simulink model "rocket_rcs"  (R2024a)
settings: Solver=FixedStepAuto  StartTime=0.0001  StopTime=140  FixedStep=0.0001  RelTol=1e-3
undefined symbols (not defined in the file or in its folder): deg, Earth, rad, s, WGS84
libraries: aerolibconvert2 x26, matrix_library x5, eePwmGenerator x5, slpidlib x5, aerolibasang x2, simulink x2, sharedtransform x1, aerolibtransform2 x1, shared6dof x1
(part 1 of 2)
settings Model: NumberOfSteps=10  Creator=WuZP  LastModifiedBy=WuZP

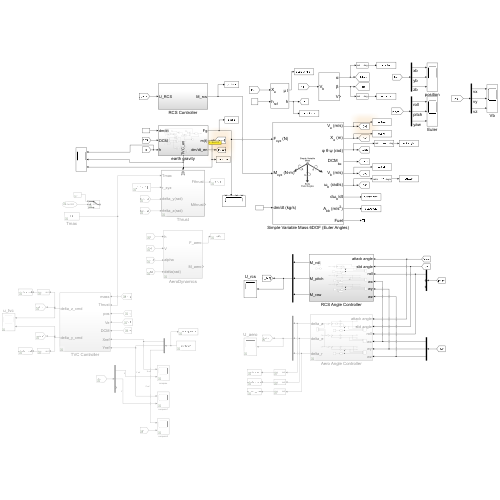
[thumbnail: Simulink's stored preview of the top-level diagram]
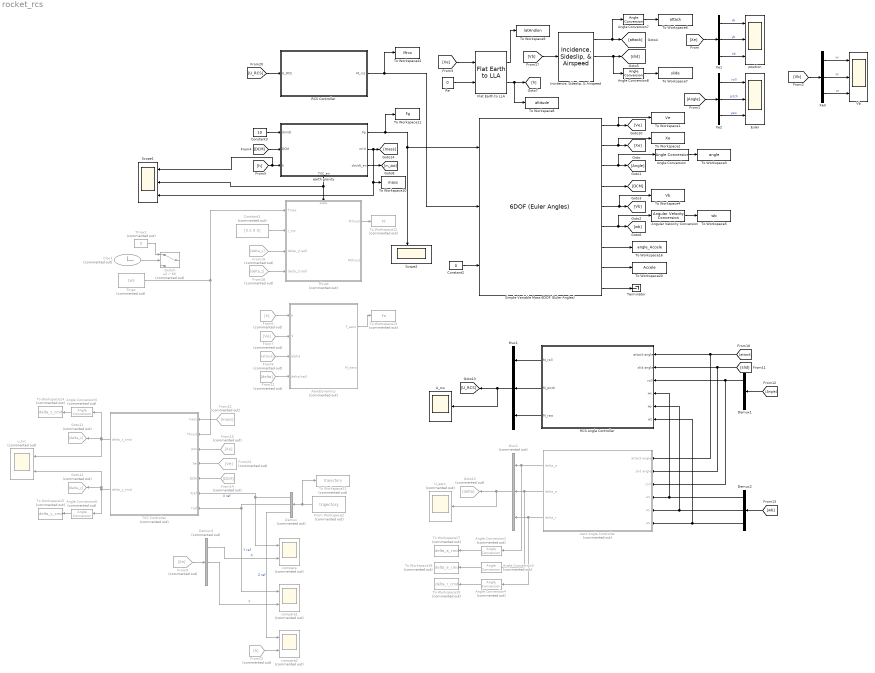
== system rocket_rcs ==
  Aero Angle Controller : Subsystem  Commented=on
  AeroDynamics : Subsystem  Commented=on
  Angle Conversion : aerolibconvert2/Angle Conversion  IU=rad  OU=deg
  Angle Conversion{2..6} (5 alike) : aerolibconvert2/Angle Conversion  Commented=on  IU=rad  OU=deg
  Angle Conversion7 : aerolibconvert2/Angle Conversion  IU=rad  OU=deg
  Angle Conversion8 : aerolibconvert2/Angle Conversion  IU=rad  OU=deg
  Angular Velocity Conversion : aerolibconvert2/Angular Velocity Conversion  IU=rad/s  OU=deg/s
  Clock : Clock  Commented=on
  Constant1 : Constant  Commented=on  Value=[3.5 0 0]
  Constant2 : Constant  Value=0
  Constant3 : Constant  Value=10
  Demux : Demux  Commented=on  Outputs=3
  Demux1 : Demux  Outputs=3
  Demux2 : Demux  Outputs=3
  Demux3 : Demux  Commented=on  Outputs=3
  Euler : Scope  NumInputPorts=3
  Flat Earth to LLA : aerolibtransform2/Flat Earth to LLA  units=Metric (MKS)  ptype=Earth (WGS84)  F=1/298.257223563  R=6378137  refPosPort=off  LL0=[39.73 98.49]  psi=0
  From Workspace2 : FromWorkspace  Commented=on  VariableName=trajectory
  From14 : From  Commented=on  GotoTag=DCM
  From15 : From  Commented=on  GotoTag=Xe
  From18 : From  Commented=on  GotoTag=delta_z
  From19 : From  Commented=on  GotoTag=delta_y
  From21 : From  Commented=on  GotoTag=mass
  From22 : From  Commented=on  GotoTag=delta
  From23 : From  Commented=on  GotoTag=h
  From24 : From  Commented=on  GotoTag=Ve
  From6 : From  Commented=on  GotoTag=h
  From7 : From  Commented=on  GotoTag=Ve
  From8 : From  Commented=on  GotoTag=attack
  From9 : From  Commented=on  GotoTag=Xe
  Goto11 : Goto  Commented=on  GotoTag=delta_z
  Goto12 : Goto  Commented=on  GotoTag=delta_y
  Goto15 : Goto  Commented=on  GotoTag=delta
  "Incidence, Sideslip, & Airspeed" : aerolibasang/Incidence, Sideslip, & Airspeed
  Mux1 : Mux  Inputs=3
  Mux2 : Mux  Commented=on  Inputs=3
  RCS Angle Controller : Subsystem
  RCS Controller : Subsystem
  Re : Constant  Value=0
  Scope1 : Scope  NumInputPorts=3
  Scope2 : Scope  NumInputPorts=4
  Simple Variable Mass 6DOF (Euler Angles) : shared6dof/6DOF (Euler Angles)  units=Metric (MKS)  mtype=Simple Variable  rep=Euler Angles  xme_0=[40719.4 121.1 -120000]  Vm_0=[7900 0 0]  eul_0=[0 0 0]  pm_0=[0 0 0]  mass_0=3600  mass_e=3600  mass_f=5000  inertia=eye(3)  inertia_e=eye(3)  inertia_f=2*eye(3)  k_quat=1.0  vre_flag=off  abi_flag=off  aMode=0  xme_statename=''  Vm_statename=''  eul_statename=''  quat_statename=''  pm_statename=''  mass_statename=''
      settings: LibrarySourceBlock=aerolib6dof2/Simple Variable Mass 6DOF (Euler Angles)
  Switch : Switch  Commented=on  Criteria=u2 > Threshold  Threshold=60  SaturateOnIntegerOverflow=off  InputSameDT=off
  TVC Controller : Subsystem  Commented=on
  Terminator : Terminator
  Thrust : Subsystem  Commented=on
  Tmax : Constant  Commented=on  Value=1e5
  Tmax1 : Constant  Commented=on  Value=0
  To Workspace1 : ToWorkspace  VariableName=Ve  SaveFormat=Timeseries  SampleTime=-1
  To Workspace10 : ToWorkspace  VariableName=mass  SaveFormat=Timeseries  SampleTime=-1
  To Workspace11 : ToWorkspace  VariableName=Fg  SaveFormat=Timeseries  SampleTime=-1
  To Workspace12 : ToWorkspace  Commented=on  VariableName=Ft  SaveFormat=Timeseries  SampleTime=-1
  To Workspace13 : ToWorkspace  Commented=on  VariableName=Fa  SaveFormat=Timeseries  SampleTime=-1
  To Workspace14 : ToWorkspace  Commented=on  VariableName=delta_z_cmd  SaveFormat=Timeseries  SampleTime=-1
  To Workspace15 : ToWorkspace  Commented=on  VariableName=delta_y_cmd  SaveFormat=Timeseries  SampleTime=-1
  To Workspace16 : ToWorkspace  VariableName=angle_Accele  SaveFormat=Timeseries  SampleTime=-1
  To Workspace17 : ToWorkspace  Commented=on  VariableName=delta_a_cmd  SaveFormat=Timeseries  SampleTime=-1
  To Workspace18 : ToWorkspace  Commented=on  VariableName=delta_e_cmd  SaveFormat=Timeseries  SampleTime=-1
  To Workspace19 : ToWorkspace  Commented=on  VariableName=delta_r_cmd  SaveFormat=Timeseries  SampleTime=-1
  To Workspace2 : ToWorkspace  VariableName=Xe  SaveFormat=Timeseries  SampleTime=-1
  To Workspace20 : ToWorkspace  VariableName=Accele  SaveFormat=Timeseries  SampleTime=-1
  To Workspace21 : ToWorkspace  Commented=on  VariableName=trajectory  SaveFormat=Timeseries  SampleTime=-1
  To Workspace22 : ToWorkspace  VariableName=Mrcs  SaveFormat=Timeseries  SampleTime=-1
  To Workspace3 : ToWorkspace  VariableName=angle  SaveFormat=Timeseries  SampleTime=-1
  To Workspace4 : ToWorkspace  VariableName=Vb  SaveFormat=Timeseries  SampleTime=-1
  To Workspace5 : ToWorkspace  VariableName=wb  SaveFormat=Timeseries  SampleTime=-1
  To Workspace6 : ToWorkspace  VariableName=attack  SaveFormat=Timeseries  SampleTime=-1
  To Workspace7 : ToWorkspace  VariableName=slide  SaveFormat=Timeseries  SampleTime=-1
  To Workspace8 : ToWorkspace  VariableName=altitude  SaveFormat=Timeseries  SampleTime=-1
  To Workspace9 : ToWorkspace  VariableName=latAndlon  SaveFormat=Timeseries  SampleTime=-1
  U_aero : Scope  Commented=on
  U_rcs : Scope
  Vb : Scope  NumInputPorts=3
  Xe1 : Demux  Outputs=3
  Xe2 : Demux  Outputs=3
  Xe3 : Demux  Outputs=3
  compare : Scope  Commented=on  NumInputPorts=2
  compare1 : Scope  Commented=on  NumInputPorts=2
  compare2 : Scope  Commented=on  NumInputPorts=2
  earth gravity : Subsystem
      settings: PortSchema="{\"entries\":[{\"content\":{\"sides\":[{\"content\":{\"connectorIds\":[\"In1\",\"In2\",\"In3\"]},\"type\":\"ConnectorPlacement.EquallySpacedRectSide\",\"uuid\":\"11dd11d9-77ad-45ee-ae63-619479f6c53b\"},{\"content\":{\"connectorIds\":[\"Out1\",\"Out2\",\"Out3\"],\"side\":\"RIGHT\"},\"type\":\"ConnectorPlacement.EquallySpacedRectSide\",\"uuid\":\"b6f331d1-51e3-4d01-85e1-3b5c4bfb552a\"},{\"content\":{\"side\":\"TOP\"},\"type\":\"ConnectorPlacement.EquallySpacedRectSide\",\"uuid\":\"4dab32ce-cfd7-4c7f-b135-3e557b532ba2\"},{\"content\":{\"connectorIds\":[\"Out4\"],\"side\":\"BOTTOM\"},\"type\":\"ConnectorPlacement.EquallySpacedRectSide\",\"uuid\":\"e34d9b96-68fb-4d6e-a900-086bc6e7115e\"}]},\"type\":\"ConnectorPlacement.EquallySpacedConnector\",\"uuid\":\"c83bfd2c-4554-412a-969b-4a26b6e2370b\"}],\"packageUris\":[\"http://schema.mathworks.com/mf0/Connector/R2020b\"],\"version\":\"1.0\"}"
  position : Scope  NumInputPorts=3
  u_tvc : Scope  Commented=on  NumInputPorts=2
  wires:
  Re/1 -> Flat Earth to LLA/2
  Tmax/1 -> Thrust/1(Tmax), TVC Controller/2(Thrust)
  Simple Variable Mass 6DOF (Euler Angles)/2 -> To Workspace2/1, [Xe]
  TVC Controller/1(delta_z_cmd) -> Angle Conversion5/1, Goto11/1, u_tvc/1
  Xe1/1 -> position/1  "xb"
  Xe1/2 -> position/2  "yb"
  Xe1/3 -> position/3  "zb"
  Simple Variable Mass 6DOF (Euler Angles)/3 -> Angle Conversion/1, [Angle]
  TVC Controller/2(delta_y_cmd) -> Goto12/1, u_tvc/2, Angle Conversion6/1
  From Workspace2/1 -> To Workspace21/1, Demux/1
  Demux/1 -> compare/1, TVC Controller/6(Xref)  "X ref"
  Demux/2 -> compare1/1, TVC Controller/7(Yref)  "Y ref"
  Constant3/1 -> earth gravity/1(dm/dt)
  Constant2/1 -> Simple Variable Mass 6DOF (Euler Angles)/3
  Simple Variable Mass 6DOF (Euler Angles)/5 -> To Workspace4/1, [Vb]
  "Incidence, Sideslip, & Airspeed"/1 -> Angle Conversion7/1, [attack]
  Xe3/3 -> Vb/3  "vz"
  Xe3/2 -> Vb/2  "vy"
  Xe3/1 -> Vb/1  "vx"
  "Incidence, Sideslip, & Airspeed"/2 -> Angle Conversion8/1, [slid]
  RCS Angle Controller/1(M_roll) -> Mux1/1
  RCS Angle Controller/2(M_pitch) -> Mux1/2
  RCS Angle Controller/3(M_raw) -> Mux1/3
  Aero Angle Controller/2(delta_e) -> Angle Conversion3/1, Mux2/2
  Aero Angle Controller/3(delta_r) -> Angle Conversion4/1, Mux2/3
  Aero Angle Controller/1(delta_a) -> Angle Conversion2/1, Mux2/1
  Mux2/1 -> Goto15/1, U_aero/1
  [Xe] -> Xe1/1
  [Vb] -> Xe3/1
  [Angle] -> Xe2/1
  Xe2/1 -> Euler/1  "roll"
  Xe2/2 -> Euler/2  "pitch"
  Xe2/3 -> Euler/3  "yaw"
  Simple Variable Mass 6DOF (Euler Angles)/4 -> [DCM]
  [Xe] -> Flat Earth to LLA/1
  Flat Earth to LLA/2 -> To Workspace8/1, [h]
  [DCM] -> earth gravity/2(DCM)
  [h] -> Scope1/1, earth gravity/3(h)
  From6/1 -> AeroDynamics/1(h)
  From7/1 -> AeroDynamics/2(V)
  From8/1 -> AeroDynamics/3(alpha)
  [attack] -> Aero Angle Controller/1(attack angle), RCS Angle Controller/1(attack angle)
  [slid] -> RCS Angle Controller/2(slid angle), Aero Angle Controller/2(slid angle)
  [Angle] -> Demux1/1
  Demux1/1 -> RCS Angle Controller/3(roll), Aero Angle Controller/3(roll)
  [wb] -> Demux2/1
  From14/1 -> TVC Controller/5(DCM)
  From15/1 -> TVC Controller/3(pos)
  Simple Variable Mass 6DOF (Euler Angles)/1 -> To Workspace1/1, [Ve]
  Constant1/1 -> Thrust/2(r_xyz)
  Simple Variable Mass 6DOF (Euler Angles)/9 -> Terminator/1
  Simple Variable Mass 6DOF (Euler Angles)/8 -> To Workspace20/1
  Simple Variable Mass 6DOF (Euler Angles)/7 -> To Workspace16/1
  [Vb] -> "Incidence, Sideslip, & Airspeed"/1
  earth gravity/4(TVC_en) -> Scope1/2, Thrust/Enable
  Mux1/1 -> [U_RCS], U_rcs/1
  [U_RCS] -> RCS Controller/1(U_RCS)
  earth gravity/2(m(t)) -> To Workspace10/1, Scope1/3, [mass]
  From21/1 -> TVC Controller/1(mass)
  From22/1 -> AeroDynamics/4(delta(rad))
  Demux2/1 -> RCS Angle Controller/4(wx), Aero Angle Controller/4(wx)
  Demux2/2 -> RCS Angle Controller/5(wy), Aero Angle Controller/5(wy)
  Demux2/3 -> RCS Angle Controller/6(wz), Aero Angle Controller/6(wz)
  Thrust/1(Fthrust) -> To Workspace12/1
  earth gravity/1(Fg) -> To Workspace11/1, Simple Variable Mass 6DOF (Euler Angles)/1, Scope2/2
  From19/1 -> Thrust/3(delta_y(rad))
  From18/1 -> Thrust/4(delta_z(rad))
  AeroDynamics/1(F_aero) -> To Workspace13/1
  From9/1 -> Demux3/1
  Demux3/1 -> compare/2  "X"
  Demux3/2 -> compare1/2  "Y"
  earth gravity/3(dm/dt_en) -> [m_dot]
  Demux/3 -> compare2/1  "Z ref"
  From23/1 -> compare2/2
  Flat Earth to LLA/1 -> To Workspace9/1
  Angle Conversion/1 -> To Workspace3/1
  Simple Variable Mass 6DOF (Euler Angles)/6 -> Angular Velocity Conversion/1, [wb]
  Angle Conversion2/1 -> To Workspace17/1
  Angle Conversion4/1 -> To Workspace19/1
  Angle Conversion3/1 -> To Workspace18/1
  Angle Conversion5/1 -> To Workspace14/1
  Angle Conversion6/1 -> To Workspace15/1
  Angle Conversion7/1 -> To Workspace6/1
  Angle Conversion8/1 -> To Workspace7/1
  Angular Velocity Conversion/1 -> To Workspace5/1
  Clock/1 -> Switch/2
  Tmax1/1 -> Switch/1
  From24/1 -> TVC Controller/4(Ve)
  RCS Controller/1(M_rcs) -> Simple Variable Mass 6DOF (Euler Angles)/2, To Workspace22/1

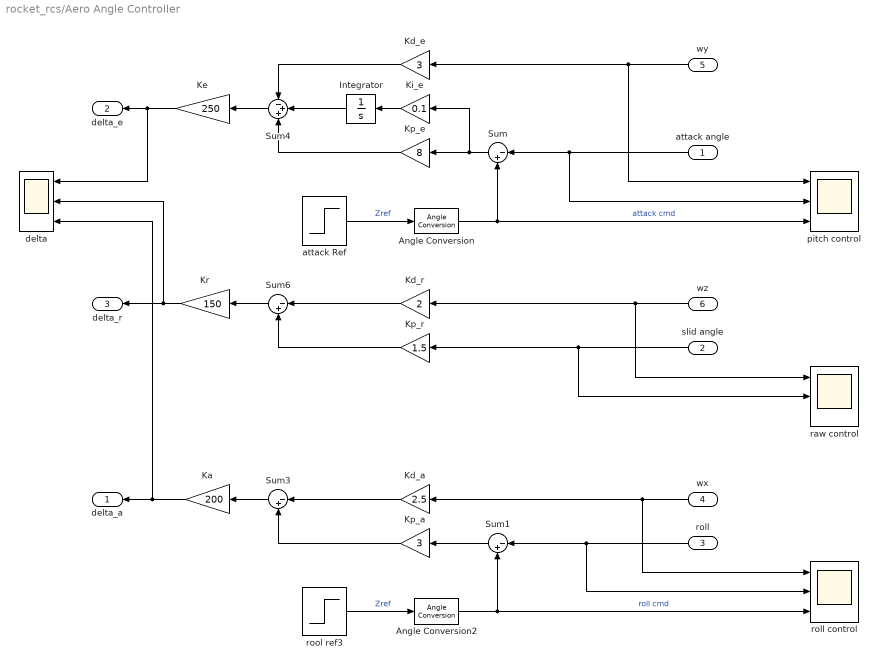
== system rocket_rcs/Aero Angle Controller ==
  attack angle : Inport
  slid angle : Inport  Port=2
  roll : Inport  Port=3
  wx : Inport  Port=4
  wy : Inport  Port=5
  wz : Inport  Port=6
  Angle Conversion : aerolibconvert2/Angle Conversion  IU=deg  OU=rad
  Angle Conversion2 : aerolibconvert2/Angle Conversion  IU=deg  OU=rad
  Integrator : Integrator
  Ka : Gain  Gain=200
  Kd_a : Gain  Gain=2.5
  Kd_e : Gain  Gain=3
  Kd_r : Gain  Gain=2
  Ke : Gain  Gain=250
  Ki_e : Gain  Gain=0.1
  Kp_a : Gain  Gain=3
  Kp_e : Gain  Gain=8
  Kp_r : Gain  Gain=1.5
  Kr : Gain  Gain=150
  Sum{,1,3,6} (4 alike) : Sum  Inputs=|-+
  Sum4 : Sum  Inputs=-++
  attack Ref : Step  After=40  SampleTime=0
  delta : Scope  NumInputPorts=3
  pitch control : Scope  NumInputPorts=3
  raw control : Scope  NumInputPorts=3
  roll control : Scope  NumInputPorts=3
  rool ref3 : Step  After=-30  SampleTime=0
  delta_a : Outport
  delta_e : Outport  Port=2
  delta_r : Outport  Port=3
  wires:
  Kp_a/1 -> Sum3/2
  Angle Conversion2/1 -> Sum1/2, roll control/3  "roll cmd"
  Angle Conversion/1 -> Sum/2, pitch control/3  "attack cmd"
  Sum/1 -> Ki_e/1, Kp_e/1
  Sum3/1 -> Ka/1
  wz/1 -> Kd_r/1, raw control/1
  wx/1 -> Kd_a/1, roll control/1
  Kp_r/1 -> Sum6/2
  Sum6/1 -> Kr/1
  Sum1/1 -> Kp_a/1
  rool ref3/1 -> Angle Conversion2/1  "Zref"
  attack Ref/1 -> Angle Conversion/1  "Zref"
  attack angle/1 -> pitch control/2, Sum/1
  wy/1 -> pitch control/1, Kd_e/1
  roll/1 -> Sum1/1, roll control/2
  Ke/1 -> delta/1, delta_e/1
  Kr/1 -> delta_r/1, delta/2
  Ka/1 -> delta/3, delta_a/1
  slid angle/1 -> Kp_r/1, raw control/2
  Ki_e/1 -> Integrator/1
  Kp_e/1 -> Sum4/3
  Kd_e/1 -> Sum4/1
  Kd_r/1 -> Sum6/1
  Kd_a/1 -> Sum3/1
  Sum4/1 -> Ke/1
  Integrator/1 -> Sum4/2

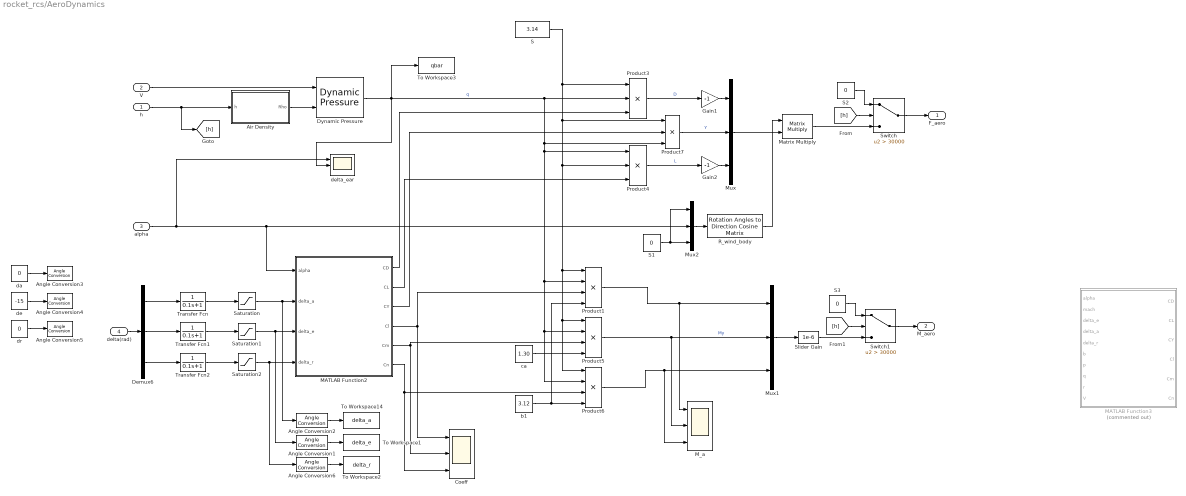
== system rocket_rcs/AeroDynamics ==
  h : Inport
  V : Inport  Port=2
  alpha : Inport  Port=3
  delta(rad) : Inport  Port=4
  Air Density : MATLAB Function  TreatAsAtomicUnit=on
  Angle Conversion1 : aerolibconvert2/Angle Conversion  IU=rad  OU=deg
  Angle Conversion2 : aerolibconvert2/Angle Conversion  IU=rad  OU=deg
  Angle Conversion3 : aerolibconvert2/Angle Conversion  IU=deg  OU=rad
  Angle Conversion4 : aerolibconvert2/Angle Conversion  IU=deg  OU=rad
  Angle Conversion5 : aerolibconvert2/Angle Conversion  IU=deg  OU=rad
  Angle Conversion6 : aerolibconvert2/Angle Conversion  IU=rad  OU=deg
  Coeff : Scope  NumInputPorts=3
  Demux6 : Demux  Outputs=3
  Dynamic Pressure : aerolibasang/Dynamic Pressure
  Gain1 : Gain  Gain=-1
  Gain2 : Gain  Gain=-1
  MATLAB Function2 : MATLAB Function  TreatAsAtomicUnit=on
  MATLAB Function3 : MATLAB Function  Commented=on  TreatAsAtomicUnit=on
  M_a : Scope  NumInputPorts=3
  Matrix Multiply : Product  Multiplication=Matrix(*)
  Mux : Mux  Inputs=3
  Mux1 : Mux  Inputs=3
  Mux2 : Mux  Inputs=3
  Product1 : Product  Inputs=4
  Product3 : Product  Inputs=3
  Product4 : Product  Inputs=3
  Product5 : Product  Inputs=4
  Product6 : Product  Inputs=4
  Product7 : Product  Inputs=3
  R_wind_body : sharedtransform/Rotation Angles to Direction Cosine Matrix  rotationOrder=XYZ  aMode=aMode
  S : Constant  Value=3.14
  S1 : Constant  Value=0
  S2 : Constant  Value=0
  S3 : Constant  Value=0
  Saturation : Saturate  UpperLimit=0.524  LowerLimit=-0.524
  Saturation1 : Saturate  UpperLimit=0.524  LowerLimit=-0.524
  Saturation2 : Saturate  UpperLimit=0.524  LowerLimit=-0.524
  Slider Gain : simulink/Math Operations/Slider Gain  gain=1e-6  low=0  high=2
  Switch : Switch  Criteria=u2 > Threshold  Threshold=30000  SaturateOnIntegerOverflow=off  InputSameDT=off
  Switch1 : Switch  Criteria=u2 > Threshold  Threshold=30000  SaturateOnIntegerOverflow=off  InputSameDT=off
  To Workspace1 : ToWorkspace  VariableName=delta_e  SaveFormat=Timeseries  SampleTime=-1
  To Workspace14 : ToWorkspace  VariableName=delta_a  SaveFormat=Timeseries  SampleTime=-1
  To Workspace2 : ToWorkspace  VariableName=delta_r  SaveFormat=Timeseries  SampleTime=-1
  To Workspace3 : ToWorkspace  VariableName=qbar  SaveFormat=Timeseries  SampleTime=-1
  Transfer Fcn : TransferFcn  Denominator=[0.1 1]
  Transfer Fcn1 : TransferFcn  Denominator=[0.1 1]
  Transfer Fcn2 : TransferFcn  Denominator=[0.1 1]
  b1 : Constant  Value=3.12
  ca : Constant  Value=1.30
  da : Constant  Value=0
  de : Constant  Value=-15
  delta_ear : Scope  NumInputPorts=3
  dr : Constant  Value=0
  F_aero : Outport
  M_aero : Outport  Port=2
  wires:
  h/1 -> [h], Air Density/1(h)
  Dynamic Pressure/1 -> To Workspace3/1, delta_ear/2, Product6/2, Product5/2, Product1/2, Product4/1, Product7/3, Product3/2  "q"
  S/1 -> Product3/1, Product7/1, Product6/1, Product5/1, Product1/1, Product4/2
  MATLAB Function2/1(CD) -> Product3/3
  MATLAB Function2/2(CL) -> Product4/3
  Mux/1 -> Matrix Multiply/2
  MATLAB Function2/5(Cm) -> Product5/3, Coeff/2
  ca/1 -> Product5/4
  Product5/1 -> M_a/2, Mux1/2  "My"
  Mux1/1 -> Slider Gain/1
  R_wind_body/1 -> Matrix Multiply/1
  alpha/1 -> delta_ear/1, MATLAB Function2/1(alpha), Mux2/2
  S1/1 -> Mux2/1, Mux2/3
  Mux2/1 -> R_wind_body/1
  Matrix Multiply/1 -> Switch/3
  Gain1/1 -> Mux/1
  Gain2/1 -> Mux/3
  Product7/1 -> Mux/2  "Y"
  Product3/1 -> Gain1/1  "D"
  Product4/1 -> Gain2/1  "L"
  Product6/1 -> M_a/3, Mux1/3
  V/1 -> Dynamic Pressure/1
  b1/1 -> Product1/4, Product6/4
  MATLAB Function2/4(Cl) -> Product1/3, Coeff/1
  MATLAB Function2/6(Cn) -> Coeff/3, Product6/3
  MATLAB Function2/3(CY) -> Product7/2
  Product1/1 -> M_a/1, Mux1/1
  Air Density/1(Rho) -> Dynamic Pressure/2
  delta(rad)/1 -> Demux6/1
  dr/1 -> Angle Conversion5/1
  de/1 -> Angle Conversion4/1
  da/1 -> Angle Conversion3/1
  Demux6/1 -> Transfer Fcn/1
  Demux6/2 -> Transfer Fcn1/1
  Demux6/3 -> Transfer Fcn2/1
  Saturation/1 -> Angle Conversion2/1, MATLAB Function2/2(delta_a)
  Saturation1/1 -> Angle Conversion1/1, MATLAB Function2/3(delta_e)
  Saturation2/1 -> Angle Conversion6/1, MATLAB Function2/4(delta_r)
  Transfer Fcn/1 -> Saturation/1
  Transfer Fcn1/1 -> Saturation1/1
  Transfer Fcn2/1 -> Saturation2/1
  [h] -> Switch/2
  S2/1 -> Switch/1
  Switch/1 -> F_aero/1
  [h] -> Switch1/2
  S3/1 -> Switch1/1
  Switch1/1 -> M_aero/1
  Slider Gain/1 -> Switch1/3
  Angle Conversion2/1 -> To Workspace14/1
  Angle Conversion1/1 -> To Workspace1/1
  Angle Conversion6/1 -> To Workspace2/1

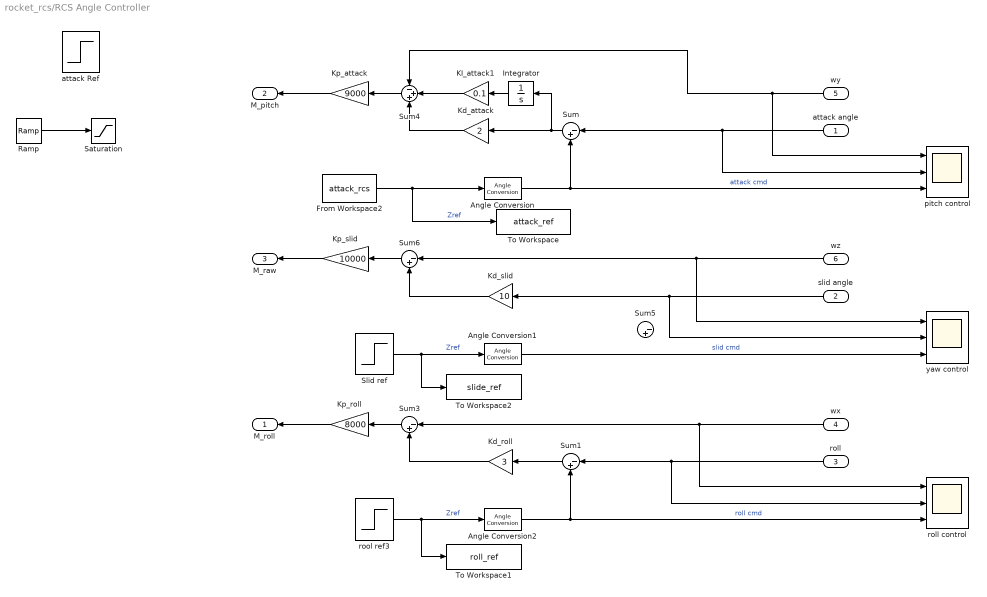
== system rocket_rcs/RCS Angle Controller ==
  attack angle : Inport
  slid angle : Inport  Port=2
  roll : Inport  Port=3
  wx : Inport  Port=4
  wy : Inport  Port=5
  wz : Inport  Port=6
  Angle Conversion : aerolibconvert2/Angle Conversion  IU=deg  OU=rad
  Angle Conversion1 : aerolibconvert2/Angle Conversion  IU=deg  OU=rad
  Angle Conversion2 : aerolibconvert2/Angle Conversion  IU=deg  OU=rad
  From Workspace2 : FromWorkspace  VariableName=attack_rcs
  Integrator : Integrator
  KI_attack1 : Gain  Gain=0.1
  Kd_attack : Gain  Gain=2
  Kd_roll : Gain  Gain=3
  Kd_slid : Gain  Gain=10
  Kp_attack : Gain  Gain=9000
  Kp_roll : Gain  Gain=8000
  Kp_slid : Gain  Gain=10000
  Ramp : simulink/Sources/Ramp  slope=2  start=5  InitialOutput=0
  Saturation : Saturate  UpperLimit=40
  Slid ref : Step  Time=0  After=0  SampleTime=0
  Sum{,1,3,5..6} (5 alike) : Sum  Inputs=|-+
  Sum4 : Sum  Inputs=-++
  To Workspace : ToWorkspace  VariableName=attack_ref  SaveFormat=Timeseries  SampleTime=-1
  To Workspace1 : ToWorkspace  VariableName=roll_ref  SaveFormat=Timeseries  SampleTime=-1
  To Workspace2 : ToWorkspace  VariableName=slide_ref  SaveFormat=Timeseries  SampleTime=-1
  attack Ref : Step  Time=5  After=40  SampleTime=0
  pitch control : Scope  NumInputPorts=3
  roll control : Scope  NumInputPorts=3
  rool ref3 : Step  Time=5  After=-70  SampleTime=0
  yaw control : Scope  NumInputPorts=3
  M_roll : Outport
  M_pitch : Outport  Port=2
  M_raw : Outport  Port=3
  wires:
  Kd_roll/1 -> Sum3/2
  Angle Conversion2/1 -> Sum1/2, roll control/3  "roll cmd"
  Angle Conversion/1 -> Sum/2, pitch control/3  "attack cmd"
  Sum/1 -> Integrator/1, Kd_attack/1
  Sum3/1 -> Kp_roll/1
  wz/1 -> yaw control/1, Sum6/1
  wx/1 -> roll control/1, Sum3/1
  Kd_slid/1 -> Sum6/2
  Sum6/1 -> Kp_slid/1
  Slid ref/1 -> Angle Conversion1/1, To Workspace2/1  "Zref"
  Angle Conversion1/1 -> yaw control/3  "slid cmd"
  Sum1/1 -> Kd_roll/1
  rool ref3/1 -> To Workspace1/1, Angle Conversion2/1  "Zref"
  Kd_attack/1 -> Sum4/3
  From Workspace2/1 -> To Workspace/1, Angle Conversion/1  "Zref"
  Sum4/1 -> Kp_attack/1
  attack angle/1 -> pitch control/2, Sum/1
  wy/1 -> pitch control/1, Sum4/1
  roll/1 -> roll control/2, Sum1/1
  Kp_attack/1 -> M_pitch/1
  Kp_slid/1 -> M_raw/1
  Kp_roll/1 -> M_roll/1
  Ramp/1 -> Saturation/1
  Integrator/1 -> KI_attack1/1
  slid angle/1 -> Kd_slid/1, yaw control/2
  KI_attack1/1 -> Sum4/2

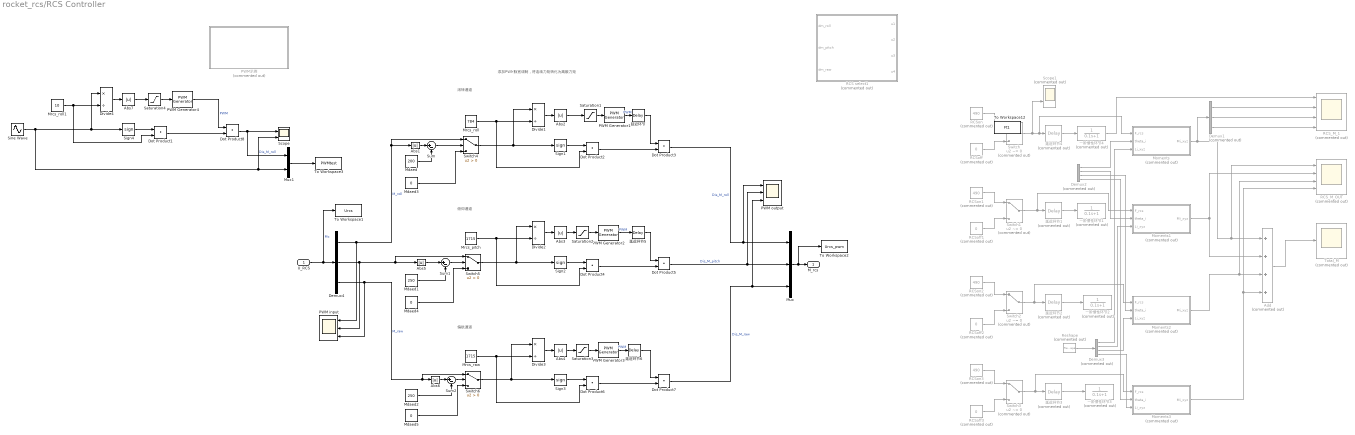
== system rocket_rcs/RCS Controller ==
  note: 添加PWM脉宽调制，将连续力矩转化为离散力矩
  note: 滚转通道
  note: 俯仰通道
  note: 偏航通道
  U_RCS : Inport
  Abs{1..7} (7 alike) : Abs  SaturateOnIntegerOverflow=off
  Add : Sum  Commented=on  Inputs=++++
  Demux1 : Demux  Commented=on  Outputs=3
  Demux2 : Demux  Commented=on
  Demux3 : Demux  Commented=on
  Demux4 : Demux  Outputs=3
  Divide{1..4} (4 alike) : Product  Inputs=*/
  Dot Product{1..8} (8 alike) : DotProduct  OutDataTypeStr=Inherit: Inherit via internal rule
  Mdaed : Constant  Value=200
  Mdaed1 : Constant  Value=250
  Mdaed2 : Constant  Value=250
  Mdaed3 : Constant  Value=0
  Mdaed4 : Constant  Value=0
  Mdaed5 : Constant  Value=0
  Moments : Subsystem  Commented=on
  Moments1 : Subsystem  Commented=on
  Moments2 : Subsystem  Commented=on
  Moments3 : Subsystem  Commented=on
  Mrcs_pitch : Constant  Value=1715
  Mrcs_raw : Constant  Value=1715
  Mrcs_roll : Constant  Value=784
  Mrcs_roll1 : Constant  Value=10
  Mux : Mux  Inputs=3
  Mux1 : Mux  Inputs=2
  PWM Generator1 : eePwmGenerator/PWM Generator  CarrCount=Up  Tper=0.1  Tdelay=0  Ts=0
  PWM Generator2 : eePwmGenerator/PWM Generator  CarrCount=Up  Tper=0.1  Tdelay=0  Ts=0
  PWM Generator3 : eePwmGenerator/PWM Generator  CarrCount=Up  Tper=0.1  Tdelay=0  Ts=0
  PWM Generator4 : eePwmGenerator/PWM Generator  CarrCount=Up  Tper=10  Tdelay=0  Ts=0
  PWM input : Scope  NumInputPorts=3
  PWM output : Scope  NumInputPorts=3
  PWM示例 : Subsystem  Commented=on
  RCS select1 : MATLAB Function  Commented=on  TreatAsAtomicUnit=on
  RCS_M_1 : Scope  Commented=on  NumInputPorts=4
  RCS_M_OUT : Scope  Commented=on  NumInputPorts=4
  RCSoff{,1..3} (4 alike) : Constant  Commented=on  Value=0
  RCSon{,1..3} (4 alike) : Constant  Commented=on  Value=490
  Reshape : Reshape  Commented=on
  Saturation{1..4} (4 alike) : Saturate  UpperLimit=1  LowerLimit=-1
  Scope : Scope  NumInputPorts=2
  Scope1 : Scope  Commented=on  NumInputPorts=2
  Sign{1..4} (4 alike) : Signum
  Sine Wave : Sin  Amplitude=10  Frequency=2*pi*0.01  SampleTime=0
  Sum : Sum  Inputs=|+-
  Sum1 : Sum  Inputs=|+-
  Sum2 : Sum  Inputs=|+-
  Switch{,1..3} (4 alike) : Switch  Commented=on  Criteria=u2 ~= 0  SaturateOnIntegerOverflow=off  InputSameDT=off
  Switch4 : Switch  Criteria=u2 > Threshold  SaturateOnIntegerOverflow=off  InputSameDT=off
  Switch5 : Switch  Criteria=u2 > Threshold  SaturateOnIntegerOverflow=off  InputSameDT=off
  Switch6 : Switch  Criteria=u2 > Threshold  SaturateOnIntegerOverflow=off  InputSameDT=off
  To Workspace1 : ToWorkspace  VariableName=Urcs  SaveFormat=Timeseries  SampleTime=-1
  To Workspace12 : ToWorkspace  VariableName=Ft1  SaveFormat=Timeseries  SampleTime=-1
  To Workspace2 : ToWorkspace  VariableName=Urcs_pwm  SaveFormat=Timeseries  SampleTime=-1
  To Workspace3 : ToWorkspace  VariableName=PWMtest  SaveFormat=Timeseries  SampleTime=-1
  Total_M : Scope  Commented=on
  一阶惯性环节{1..4} (4 alike) : TransferFcn  Commented=on  Denominator=[0.1 1]
  延迟环节 : TransportDelay  DelayTime=0.001
  延迟环节{1..4} (4 alike) : TransportDelay  Commented=on  DelayTime=0
  延迟环节5 : TransportDelay  DelayTime=0.001
  延迟环节6 : TransportDelay  DelayTime=0.001
  M_rcs : Outport
  wires:
  RCSon/1 -> Switch/1
  RCSoff/1 -> Switch/3
  Switch1/1 -> Moments1/1(F_rcs), 延迟环节1/1
  Moments1/1(Mi_xyz) -> RCS_M_OUT/2, Add/2
  延迟环节1/1 -> 一阶惯性环节1/1
  RCSon1/1 -> Switch1/1
  RCSoff1/1 -> Switch1/3
  Switch2/1 -> Moments2/1(F_rcs), 延迟环节2/1
  Moments2/1(Mi_xyz) -> RCS_M_OUT/3, Add/3
  延迟环节2/1 -> 一阶惯性环节2/1
  RCSon2/1 -> Switch2/1
  RCSoff2/1 -> Switch2/3
  Switch3/1 -> Moments3/1(F_rcs), 延迟环节3/1
  Moments3/1(Mi_xyz) -> RCS_M_OUT/4, Add/4
  延迟环节3/1 -> 一阶惯性环节3/1
  RCSon3/1 -> Switch3/1
  RCSoff3/1 -> Switch3/3
  Moments/1(Mi_xyz) -> Demux1/1, RCS_M_OUT/1, Add/1
  Demux1/1 -> RCS_M_1/2
  Demux1/2 -> RCS_M_1/3
  Demux1/3 -> RCS_M_1/4
  Switch/1 -> Moments/1(F_rcs), 延迟环节4/1, Scope1/2
  延迟环节4/1 -> 一阶惯性环节4/1
  一阶惯性环节4/1 -> RCS_M_1/1
  Add/1 -> Total_M/1
  Demux2/1 -> Moments/2(theta_i)
  Demux2/2 -> Moments1/2(theta_i)
  Demux2/3 -> Moments2/2(theta_i)
  Demux2/4 -> Moments3/2(theta_i)
  Demux3/1 -> Moments/3(Li_xyz)
  Demux3/2 -> Moments1/3(Li_xyz)
  Demux3/3 -> Moments2/3(Li_xyz)
  Demux3/4 -> Moments3/3(Li_xyz)
  Reshape/1 -> Demux3/1
  Divide1/1 -> Abs2/1
  Abs2/1 -> Saturation1/1
  Saturation1/1 -> PWM Generator1/1
  PWM Generator1/1 -> 延迟环节/1  "PWM"
  Sign1/1 -> Dot Product2/1
  Mrcs_roll/1 -> Dot Product2/2, Divide1/2
  Dot Product2/1 -> Dot Product3/2
  U_RCS/1 -> To Workspace1/1, Demux4/1  "Mc"
  Dot Product5/1 -> Mux/2, PWM output/2  "Dis_M_pitch"
  Saturation2/1 -> PWM Generator2/1
  Abs3/1 -> Saturation2/1
  Mrcs_pitch/1 -> Dot Product4/2, Divide2/2
  Dot Product4/1 -> Dot Product5/2
  Divide2/1 -> Abs3/1
  Sign2/1 -> Dot Product4/1
  PWM Generator2/1 -> 延迟环节5/1  "PWM"
  Dot Product7/1 -> PWM output/3, Mux/3  "Dis_M_raw"
  Saturation3/1 -> PWM Generator3/1
  Abs4/1 -> Saturation3/1
  Mrcs_raw/1 -> Dot Product6/2, Divide3/2
  Dot Product6/1 -> Dot Product7/2
  Divide3/1 -> Abs4/1
  Sign3/1 -> Dot Product6/1
  PWM Generator3/1 -> 延迟环节6/1  "PWM"
  Demux4/3 -> Switch6/1, Abs6/1, PWM input/3  "M_raw"
  Dot Product3/1 -> PWM output/1, Mux/1  "Dis_M_roll"
  Mux/1 -> To Workspace2/1, M_rcs/1
  Demux4/1 -> Abs1/1, Switch4/1, PWM input/1  "M_roll"
  Demux4/2 -> Abs5/1, Switch5/1, PWM input/2
  Switch4/1 -> Divide1/1, Sign1/1
  Switch5/1 -> Divide2/1, Sign2/1
  Switch6/1 -> Divide3/1, Sign3/1
  Sum/1 -> Switch4/2
  Mdaed/1 -> Sum/2
  Mdaed1/1 -> Sum1/2
  Sum1/1 -> Switch5/2
  Mdaed2/1 -> Sum2/2
  Sum2/1 -> Switch6/2
  Mdaed3/1 -> Switch4/3
  Mdaed4/1 -> Switch5/3
  Mdaed5/1 -> Switch6/3
  Abs1/1 -> Sum/1
  Abs5/1 -> Sum1/1
  Abs6/1 -> Sum2/1
  延迟环节/1 -> Dot Product3/1
  延迟环节5/1 -> Dot Product5/1
  延迟环节6/1 -> Dot Product7/1
  Divide4/1 -> Abs7/1
  Saturation4/1 -> PWM Generator4/1
  Dot Product1/1 -> Dot Product8/2
  Sign4/1 -> Dot Product1/1
  Abs7/1 -> Saturation4/1
  PWM Generator4/1 -> Dot Product8/1  "PWM"
  Mrcs_roll1/1 -> Dot Product1/2, Divide4/2
  Sine Wave/1 -> Scope/2, Mux1/2, Divide4/1, Sign4/1
  Dot Product8/1 -> Scope/1, Mux1/1  "Dis_M_roll"
  Mux1/1 -> To Workspace3/1

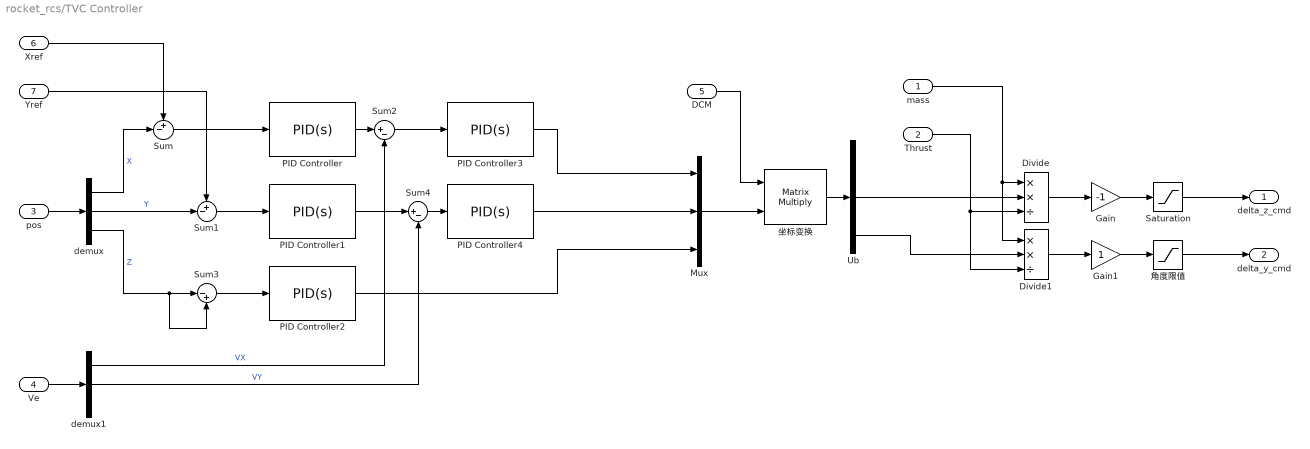
== system rocket_rcs/TVC Controller ==
  mass : Inport
  Thrust : Inport  Port=2
  pos : Inport  Port=3
  Ve : Inport  Port=4
  DCM : Inport  Port=5
  Xref : Inport  Port=6
  Yref : Inport  Port=7
  Divide : Product  Inputs=**/
  Divide1 : Product  Inputs=**/
  Gain : Gain  Gain=-1
  Gain1 : Gain
  Mux : Mux  Inputs=3
  PID Controller : slpidlib/PID Controller  Controller=PID  Form=Parallel  TimeDomain=Continuous-time  UseExternalTs=off  SampleTime=-1  IntegratorMethod=Forward Euler  FilterMethod=Forward Euler  ControllerParametersSource=internal  P=10  I=0  UseKiTs=off  D=8  UseExternalDerivativeSource=off  N=100  UseFilter=on  TunerSelectOption=Transfer Function Based (PID Tuner App)  InitialConditionSource=internal  InitialConditionForIntegrator=0  InitialConditionForFilter=0  DifferentiatorICPrevScaledInput=0  ExternalReset=none  TrackingMode=off  Kt=1  LimitOutput=off  SatLimitsSource=internal  UpperSaturationLimit=inf  LowerSaturationLimit=-inf  LinearizeAsGain=on  AntiWindupMode=none  Kb=1  LimitIntegrator=off  UpperIntegratorSaturationLimit=inf  LowerIntegratorSaturationLimit=-inf  POutMin=[]  POutMax=[]  IOutMin=[]  IOutMax=[]  DOutMin=[]  DOutMax=[]  NOutMin=[]  NOutMax=[]  SumOutMin=[]  SumOutMax=[]  SaturationOutMin=[]  SaturationOutMax=[]  PParamMin=[]  PParamMax=[]  IParamMin=[]  IParamMax=[]  DParamMin=[]  DParamMax=[]  NParamMin=[]  NParamMax=[]  KbParamMin=[]  KbParamMax=[]  KtParamMin=[]  KtParamMax=[]  KbOutMin=[]  KbOutMax=[]  KtOutMin=[]  KtOutMax=[]  IntegratorOutMin=[]  IntegratorOutMax=[]  FilterOutMin=[]  FilterOutMax=[]  SumI1OutMin=[]  SumI1OutMax=[]  SumI2OutMin=[]  SumI2OutMax=[]  SumI3OutMin=[]  SumI3OutMax=[]  SumI4OutMin=[]  SumI4OutMax=[]  SumDOutMin=[]  SumDOutMax=[]  DifferentiatorOutMin=[]  DifferentiatorOutMax=[]  FilterDiffOutCoefMin=[]  FilterDiffOutCoefMax=[]  ReciprocalOutMin=[]  ReciprocalOutMax=[]  SumDenOutMin=[]  SumDenOutMax=[]  SumNumOutMin=[]  SumNumOutMax=[]  DivideOutMin=[]  DivideOutMax=[]  UdiffTsProdOutMin=[]  UdiffTsProdOutMax=[]  NTsProdOutMin=[]  NTsProdOutMax=[]  UintegralTsProdOutMin=[]  UintegralTsProdOutMax=[]  UngainTsProdOutMin=[]  UngainTsProdOutMax=[]  ClampingZeroOutDataTypeStr=Inherit: Inherit via back propagation  ClampingZeroOutMin=[]  ClampingZeroOutMax=[]  FilterDenConstantOutDataTypeStr=Inherit: Inherit via back propagation  FilterDenConstantOutMin=[]  FilterDenConstantOutMax=[]  PCopyOutDataTypeStr=Inherit: Inherit via back propagation  PCopyOutMin=[]  PCopyOutMax=[]  NCopyOutDataTypeStr=Inherit: Inherit via back propagation  NCopyOutMin=[]  NCopyOutMax=[]  IntegratorContinuousStateAttributes=''  IntegratorStateMustResolveToSignalObject=off  IntegratorRTWStateStorageClass=Auto  FilterContinuousStateAttributes=''  FilterStateMustResolveToSignalObject=off  FilterRTWStateStorageClass=Auto  ParallelPVariant=InternalParameters  IdealPVariant=Disabled  IVariant=InternalParameters  DVariant=InternalParameters  IntegratorVariant=Continuous  SatVariant=Disabled  AWVariant=Passthrough  PCopyVariant=Disabled  TRVariant=Disabled  FdbkBlocksVariant=Forward  IdealPFdbkVariant=Disabled  SatFdbkVariant=Disabled  DerivativeFilterVariant=ContFilter  NVariant=InternalParameters  NCopyVariant=Disabled  FilterICVariant=InternalICsFilter  IntegratorICVariant=InternalICs  ExternalResetVariant=Disabled  TRSumVariant=Passthrough  SumFdbkVariant=Disabled  SumVariant=Sum_PID  TsampFilterVariant=InternalTs  TsampNgainVariant=Passthrough  TsampIntegralVariant=Disabled_SignalSpec  ExternalSaturationOutDataTypeStr=Inherit: Same as second input  DerivativeSourceVariant=ErrorSignal
  PID Controller1 : slpidlib/PID Controller  Controller=PID  Form=Parallel  TimeDomain=Continuous-time  UseExternalTs=off  SampleTime=-1  IntegratorMethod=Forward Euler  FilterMethod=Forward Euler  ControllerParametersSource=internal  P=5  I=0  UseKiTs=off  D=8  UseExternalDerivativeSource=off  N=100  UseFilter=on  TunerSelectOption=Transfer Function Based (PID Tuner App)  InitialConditionSource=internal  InitialConditionForIntegrator=0  InitialConditionForFilter=0  DifferentiatorICPrevScaledInput=0  ExternalReset=none  TrackingMode=off  Kt=1  LimitOutput=off  SatLimitsSource=internal  UpperSaturationLimit=inf  LowerSaturationLimit=-inf  LinearizeAsGain=on  AntiWindupMode=none  Kb=1  LimitIntegrator=off  UpperIntegratorSaturationLimit=inf  LowerIntegratorSaturationLimit=-inf  POutMin=[]  POutMax=[]  IOutMin=[]  IOutMax=[]  DOutMin=[]  DOutMax=[]  NOutMin=[]  NOutMax=[]  SumOutMin=[]  SumOutMax=[]  SaturationOutMin=[]  SaturationOutMax=[]  PParamMin=[]  PParamMax=[]  IParamMin=[]  IParamMax=[]  DParamMin=[]  DParamMax=[]  NParamMin=[]  NParamMax=[]  KbParamMin=[]  KbParamMax=[]  KtParamMin=[]  KtParamMax=[]  KbOutMin=[]  KbOutMax=[]  KtOutMin=[]  KtOutMax=[]  IntegratorOutMin=[]  IntegratorOutMax=[]  FilterOutMin=[]  FilterOutMax=[]  SumI1OutMin=[]  SumI1OutMax=[]  SumI2OutMin=[]  SumI2OutMax=[]  SumI3OutMin=[]  SumI3OutMax=[]  SumI4OutMin=[]  SumI4OutMax=[]  SumDOutMin=[]  SumDOutMax=[]  DifferentiatorOutMin=[]  DifferentiatorOutMax=[]  FilterDiffOutCoefMin=[]  FilterDiffOutCoefMax=[]  ReciprocalOutMin=[]  ReciprocalOutMax=[]  SumDenOutMin=[]  SumDenOutMax=[]  SumNumOutMin=[]  SumNumOutMax=[]  DivideOutMin=[]  DivideOutMax=[]  UdiffTsProdOutMin=[]  UdiffTsProdOutMax=[]  NTsProdOutMin=[]  NTsProdOutMax=[]  UintegralTsProdOutMin=[]  UintegralTsProdOutMax=[]  UngainTsProdOutMin=[]  UngainTsProdOutMax=[]  ClampingZeroOutDataTypeStr=Inherit: Inherit via back propagation  ClampingZeroOutMin=[]  ClampingZeroOutMax=[]  FilterDenConstantOutDataTypeStr=Inherit: Inherit via back propagation  FilterDenConstantOutMin=[]  FilterDenConstantOutMax=[]  PCopyOutDataTypeStr=Inherit: Inherit via back propagation  PCopyOutMin=[]  PCopyOutMax=[]  NCopyOutDataTypeStr=Inherit: Inherit via back propagation  NCopyOutMin=[]  NCopyOutMax=[]  IntegratorContinuousStateAttributes=''  IntegratorStateMustResolveToSignalObject=off  IntegratorRTWStateStorageClass=Auto  FilterContinuousStateAttributes=''  FilterStateMustResolveToSignalObject=off  FilterRTWStateStorageClass=Auto  ParallelPVariant=InternalParameters  IdealPVariant=Disabled  IVariant=InternalParameters  DVariant=InternalParameters  IntegratorVariant=Continuous  SatVariant=Disabled  AWVariant=Passthrough  PCopyVariant=Disabled  TRVariant=Disabled  FdbkBlocksVariant=Forward  IdealPFdbkVariant=Disabled  SatFdbkVariant=Disabled  DerivativeFilterVariant=ContFilter  NVariant=InternalParameters  NCopyVariant=Disabled  FilterICVariant=InternalICsFilter  IntegratorICVariant=InternalICs  ExternalResetVariant=Disabled  TRSumVariant=Passthrough  SumFdbkVariant=Disabled  SumVariant=Sum_PID  TsampFilterVariant=InternalTs  TsampNgainVariant=Passthrough  TsampIntegralVariant=Disabled_SignalSpec  ExternalSaturationOutDataTypeStr=Inherit: Same as second input  DerivativeSourceVariant=ErrorSignal
  PID Controller2 : slpidlib/PID Controller  Controller=PID  Form=Parallel  TimeDomain=Continuous-time  UseExternalTs=off  SampleTime=-1  IntegratorMethod=Forward Euler  FilterMethod=Forward Euler  ControllerParametersSource=internal  P=8  I=0.5  UseKiTs=off  D=8  UseExternalDerivativeSource=off  N=100  UseFilter=on  TunerSelectOption=Transfer Function Based (PID Tuner App)  InitialConditionSource=internal  InitialConditionForIntegrator=0  InitialConditionForFilter=0  DifferentiatorICPrevScaledInput=0  ExternalReset=none  TrackingMode=off  Kt=1  LimitOutput=off  SatLimitsSource=internal  UpperSaturationLimit=inf  LowerSaturationLimit=-inf  LinearizeAsGain=on  AntiWindupMode=none  Kb=1  LimitIntegrator=off  UpperIntegratorSaturationLimit=inf  LowerIntegratorSaturationLimit=-inf  POutMin=[]  POutMax=[]  IOutMin=[]  IOutMax=[]  DOutMin=[]  DOutMax=[]  NOutMin=[]  NOutMax=[]  SumOutMin=[]  SumOutMax=[]  SaturationOutMin=[]  SaturationOutMax=[]  PParamMin=[]  PParamMax=[]  IParamMin=[]  IParamMax=[]  DParamMin=[]  DParamMax=[]  NParamMin=[]  NParamMax=[]  KbParamMin=[]  KbParamMax=[]  KtParamMin=[]  KtParamMax=[]  KbOutMin=[]  KbOutMax=[]  KtOutMin=[]  KtOutMax=[]  IntegratorOutMin=[]  IntegratorOutMax=[]  FilterOutMin=[]  FilterOutMax=[]  SumI1OutMin=[]  SumI1OutMax=[]  SumI2OutMin=[]  SumI2OutMax=[]  SumI3OutMin=[]  SumI3OutMax=[]  SumI4OutMin=[]  SumI4OutMax=[]  SumDOutMin=[]  SumDOutMax=[]  DifferentiatorOutMin=[]  DifferentiatorOutMax=[]  FilterDiffOutCoefMin=[]  FilterDiffOutCoefMax=[]  ReciprocalOutMin=[]  ReciprocalOutMax=[]  SumDenOutMin=[]  SumDenOutMax=[]  SumNumOutMin=[]  SumNumOutMax=[]  DivideOutMin=[]  DivideOutMax=[]  UdiffTsProdOutMin=[]  UdiffTsProdOutMax=[]  NTsProdOutMin=[]  NTsProdOutMax=[]  UintegralTsProdOutMin=[]  UintegralTsProdOutMax=[]  UngainTsProdOutMin=[]  UngainTsProdOutMax=[]  ClampingZeroOutDataTypeStr=Inherit: Inherit via back propagation  ClampingZeroOutMin=[]  ClampingZeroOutMax=[]  FilterDenConstantOutDataTypeStr=Inherit: Inherit via back propagation  FilterDenConstantOutMin=[]  FilterDenConstantOutMax=[]  PCopyOutDataTypeStr=Inherit: Inherit via back propagation  PCopyOutMin=[]  PCopyOutMax=[]  NCopyOutDataTypeStr=Inherit: Inherit via back propagation  NCopyOutMin=[]  NCopyOutMax=[]  IntegratorContinuousStateAttributes=''  IntegratorStateMustResolveToSignalObject=off  IntegratorRTWStateStorageClass=Auto  FilterContinuousStateAttributes=''  FilterStateMustResolveToSignalObject=off  FilterRTWStateStorageClass=Auto  ParallelPVariant=InternalParameters  IdealPVariant=Disabled  IVariant=InternalParameters  DVariant=InternalParameters  IntegratorVariant=Continuous  SatVariant=Disabled  AWVariant=Passthrough  PCopyVariant=Disabled  TRVariant=Disabled  FdbkBlocksVariant=Forward  IdealPFdbkVariant=Disabled  SatFdbkVariant=Disabled  DerivativeFilterVariant=ContFilter  NVariant=InternalParameters  NCopyVariant=Disabled  FilterICVariant=InternalICsFilter  IntegratorICVariant=InternalICs  ExternalResetVariant=Disabled  TRSumVariant=Passthrough  SumFdbkVariant=Disabled  SumVariant=Sum_PID  TsampFilterVariant=InternalTs  TsampNgainVariant=Passthrough  TsampIntegralVariant=Disabled_SignalSpec  ExternalSaturationOutDataTypeStr=Inherit: Same as second input  DerivativeSourceVariant=ErrorSignal
  PID Controller3 : slpidlib/PID Controller  Controller=PID  Form=Parallel  TimeDomain=Continuous-time  UseExternalTs=off  SampleTime=-1  IntegratorMethod=Forward Euler  FilterMethod=Forward Euler  ControllerParametersSource=internal  P=10  I=0  UseKiTs=off  D=8  UseExternalDerivativeSource=off  N=100  UseFilter=on  TunerSelectOption=Transfer Function Based (PID Tuner App)  InitialConditionSource=internal  InitialConditionForIntegrator=0  InitialConditionForFilter=0  DifferentiatorICPrevScaledInput=0  ExternalReset=none  TrackingMode=off  Kt=1  LimitOutput=off  SatLimitsSource=internal  UpperSaturationLimit=inf  LowerSaturationLimit=-inf  LinearizeAsGain=on  AntiWindupMode=none  Kb=1  LimitIntegrator=off  UpperIntegratorSaturationLimit=inf  LowerIntegratorSaturationLimit=-inf  POutMin=[]  POutMax=[]  IOutMin=[]  IOutMax=[]  DOutMin=[]  DOutMax=[]  NOutMin=[]  NOutMax=[]  SumOutMin=[]  SumOutMax=[]  SaturationOutMin=[]  SaturationOutMax=[]  PParamMin=[]  PParamMax=[]  IParamMin=[]  IParamMax=[]  DParamMin=[]  DParamMax=[]  NParamMin=[]  NParamMax=[]  KbParamMin=[]  KbParamMax=[]  KtParamMin=[]  KtParamMax=[]  KbOutMin=[]  KbOutMax=[]  KtOutMin=[]  KtOutMax=[]  IntegratorOutMin=[]  IntegratorOutMax=[]  FilterOutMin=[]  FilterOutMax=[]  SumI1OutMin=[]  SumI1OutMax=[]  SumI2OutMin=[]  SumI2OutMax=[]  SumI3OutMin=[]  SumI3OutMax=[]  SumI4OutMin=[]  SumI4OutMax=[]  SumDOutMin=[]  SumDOutMax=[]  DifferentiatorOutMin=[]  DifferentiatorOutMax=[]  FilterDiffOutCoefMin=[]  FilterDiffOutCoefMax=[]  ReciprocalOutMin=[]  ReciprocalOutMax=[]  SumDenOutMin=[]  SumDenOutMax=[]  SumNumOutMin=[]  SumNumOutMax=[]  DivideOutMin=[]  DivideOutMax=[]  UdiffTsProdOutMin=[]  UdiffTsProdOutMax=[]  NTsProdOutMin=[]  NTsProdOutMax=[]  UintegralTsProdOutMin=[]  UintegralTsProdOutMax=[]  UngainTsProdOutMin=[]  UngainTsProdOutMax=[]  ClampingZeroOutDataTypeStr=Inherit: Inherit via back propagation  ClampingZeroOutMin=[]  ClampingZeroOutMax=[]  FilterDenConstantOutDataTypeStr=Inherit: Inherit via back propagation  FilterDenConstantOutMin=[]  FilterDenConstantOutMax=[]  PCopyOutDataTypeStr=Inherit: Inherit via back propagation  PCopyOutMin=[]  PCopyOutMax=[]  NCopyOutDataTypeStr=Inherit: Inherit via back propagation  NCopyOutMin=[]  NCopyOutMax=[]  IntegratorContinuousStateAttributes=''  IntegratorStateMustResolveToSignalObject=off  IntegratorRTWStateStorageClass=Auto  FilterContinuousStateAttributes=''  FilterStateMustResolveToSignalObject=off  FilterRTWStateStorageClass=Auto  ParallelPVariant=InternalParameters  IdealPVariant=Disabled  IVariant=InternalParameters  DVariant=InternalParameters  IntegratorVariant=Continuous  SatVariant=Disabled  AWVariant=Passthrough  PCopyVariant=Disabled  TRVariant=Disabled  FdbkBlocksVariant=Forward  IdealPFdbkVariant=Disabled  SatFdbkVariant=Disabled  DerivativeFilterVariant=ContFilter  NVariant=InternalParameters  NCopyVariant=Disabled  FilterICVariant=InternalICsFilter  IntegratorICVariant=InternalICs  ExternalResetVariant=Disabled  TRSumVariant=Passthrough  SumFdbkVariant=Disabled  SumVariant=Sum_PID  TsampFilterVariant=InternalTs  TsampNgainVariant=Passthrough  TsampIntegralVariant=Disabled_SignalSpec  ExternalSaturationOutDataTypeStr=Inherit: Same as second input  DerivativeSourceVariant=ErrorSignal
  PID Controller4 : slpidlib/PID Controller  Controller=PID  Form=Parallel  TimeDomain=Continuous-time  UseExternalTs=off  SampleTime=-1  IntegratorMethod=Forward Euler  FilterMethod=Forward Euler  ControllerParametersSource=internal  P=5  I=0  UseKiTs=off  D=8  UseExternalDerivativeSource=off  N=100  UseFilter=on  TunerSelectOption=Transfer Function Based (PID Tuner App)  InitialConditionSource=internal  InitialConditionForIntegrator=0  InitialConditionForFilter=0  DifferentiatorICPrevScaledInput=0  ExternalReset=none  TrackingMode=off  Kt=1  LimitOutput=off  SatLimitsSource=internal  UpperSaturationLimit=inf  LowerSaturationLimit=-inf  LinearizeAsGain=on  AntiWindupMode=none  Kb=1  LimitIntegrator=off  UpperIntegratorSaturationLimit=inf  LowerIntegratorSaturationLimit=-inf  POutMin=[]  POutMax=[]  IOutMin=[]  IOutMax=[]  DOutMin=[]  DOutMax=[]  NOutMin=[]  NOutMax=[]  SumOutMin=[]  SumOutMax=[]  SaturationOutMin=[]  SaturationOutMax=[]  PParamMin=[]  PParamMax=[]  IParamMin=[]  IParamMax=[]  DParamMin=[]  DParamMax=[]  NParamMin=[]  NParamMax=[]  KbParamMin=[]  KbParamMax=[]  KtParamMin=[]  KtParamMax=[]  KbOutMin=[]  KbOutMax=[]  KtOutMin=[]  KtOutMax=[]  IntegratorOutMin=[]  IntegratorOutMax=[]  FilterOutMin=[]  FilterOutMax=[]  SumI1OutMin=[]  SumI1OutMax=[]  SumI2OutMin=[]  SumI2OutMax=[]  SumI3OutMin=[]  SumI3OutMax=[]  SumI4OutMin=[]  SumI4OutMax=[]  SumDOutMin=[]  SumDOutMax=[]  DifferentiatorOutMin=[]  DifferentiatorOutMax=[]  FilterDiffOutCoefMin=[]  FilterDiffOutCoefMax=[]  ReciprocalOutMin=[]  ReciprocalOutMax=[]  SumDenOutMin=[]  SumDenOutMax=[]  SumNumOutMin=[]  SumNumOutMax=[]  DivideOutMin=[]  DivideOutMax=[]  UdiffTsProdOutMin=[]  UdiffTsProdOutMax=[]  NTsProdOutMin=[]  NTsProdOutMax=[]  UintegralTsProdOutMin=[]  UintegralTsProdOutMax=[]  UngainTsProdOutMin=[]  UngainTsProdOutMax=[]  ClampingZeroOutDataTypeStr=Inherit: Inherit via back propagation  ClampingZeroOutMin=[]  ClampingZeroOutMax=[]  FilterDenConstantOutDataTypeStr=Inherit: Inherit via back propagation  FilterDenConstantOutMin=[]  FilterDenConstantOutMax=[]  PCopyOutDataTypeStr=Inherit: Inherit via back propagation  PCopyOutMin=[]  PCopyOutMax=[]  NCopyOutDataTypeStr=Inherit: Inherit via back propagation  NCopyOutMin=[]  NCopyOutMax=[]  IntegratorContinuousStateAttributes=''  IntegratorStateMustResolveToSignalObject=off  IntegratorRTWStateStorageClass=Auto  FilterContinuousStateAttributes=''  FilterStateMustResolveToSignalObject=off  FilterRTWStateStorageClass=Auto  ParallelPVariant=InternalParameters  IdealPVariant=Disabled  IVariant=InternalParameters  DVariant=InternalParameters  IntegratorVariant=Continuous  SatVariant=Disabled  AWVariant=Passthrough  PCopyVariant=Disabled  TRVariant=Disabled  FdbkBlocksVariant=Forward  IdealPFdbkVariant=Disabled  SatFdbkVariant=Disabled  DerivativeFilterVariant=ContFilter  NVariant=InternalParameters  NCopyVariant=Disabled  FilterICVariant=InternalICsFilter  IntegratorICVariant=InternalICs  ExternalResetVariant=Disabled  TRSumVariant=Passthrough  SumFdbkVariant=Disabled  SumVariant=Sum_PID  TsampFilterVariant=InternalTs  TsampNgainVariant=Passthrough  TsampIntegralVariant=Disabled_SignalSpec  ExternalSaturationOutDataTypeStr=Inherit: Same as second input  DerivativeSourceVariant=ErrorSignal
  Saturation : Saturate  UpperLimit=0.349  LowerLimit=-0.349
  Sum : Sum  Inputs=+-|
  Sum1 : Sum  Inputs=+-|
  Sum2 : Sum  Inputs=|+-
  Sum3 : Sum  Inputs=|-+
  Sum4 : Sum  Inputs=|+-
  Ub : Demux  Outputs=3
  demux : Demux  Outputs=3
  demux1 : Demux  Outputs=3
  坐标变换 : Product  Multiplication=Matrix(*)
  角度限值 : Saturate  UpperLimit=0.349  LowerLimit=-0.349
  delta_z_cmd : Outport
  delta_y_cmd : Outport  Port=2
  wires:
  DCM/1 -> 坐标变换/1
  Divide/1 -> Gain/1
  Sum/1 -> PID Controller/1
  PID Controller/1 -> Sum2/1
  Sum1/1 -> PID Controller1/1
  mass/1 -> Divide1/1, Divide/1
  Thrust/1 -> Divide1/3, Divide/3
  PID Controller1/1 -> Sum4/1
  demux/3 -> Sum3/1, Sum3/2  "Z"
  Divide1/1 -> Gain1/1
  Ub/3 -> Divide1/2
  Ub/2 -> Divide/2
  Gain/1 -> Saturation/1
  Mux/1 -> 坐标变换/2
  坐标变换/1 -> Ub/1
  Sum3/1 -> PID Controller2/1
  pos/1 -> demux/1
  Gain1/1 -> 角度限值/1
  Xref/1 -> Sum/1
  demux/1 -> Sum/2  "X"
  Yref/1 -> Sum1/1
  demux/2 -> Sum1/2  "Y"
  Saturation/1 -> delta_z_cmd/1
  角度限值/1 -> delta_y_cmd/1
  Ve/1 -> demux1/1
  Sum2/1 -> PID Controller3/1
  demux1/1 -> Sum2/2  "VX"
  Sum4/1 -> PID Controller4/1
  demux1/2 -> Sum4/2  "VY"
  PID Controller3/1 -> Mux/1
  PID Controller4/1 -> Mux/2
  PID Controller2/1 -> Mux/3

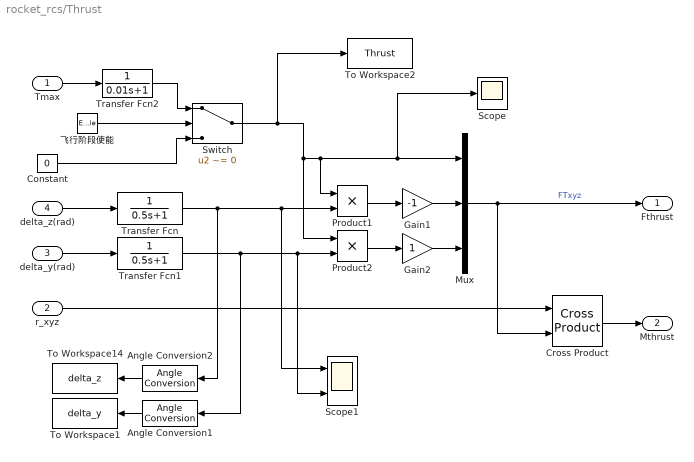
== system rocket_rcs/Thrust ==
  Tmax : Inport
  r_xyz : Inport  Port=2
  delta_y(rad) : Inport  Port=3
  delta_z(rad) : Inport  Port=4
  飞行阶段使能 : EnablePort  StatesWhenEnabling=reset  ShowOutputPort=on
  Angle Conversion1 : aerolibconvert2/Angle Conversion  IU=rad  OU=deg
  Angle Conversion2 : aerolibconvert2/Angle Conversion  IU=rad  OU=deg
  Constant : Constant  Value=0
  Cross Product : matrix_library/Cross Product
  Gain1 : Gain  Gain=-1
  Gain2 : Gain
  Mux : Mux  Inputs=3
  Product1 : Product
  Product2 : Product
  Scope : Scope
  Scope1 : Scope  NumInputPorts=2
  Switch : Switch  Criteria=u2 ~= 0  SaturateOnIntegerOverflow=off  InputSameDT=off
  To Workspace1 : ToWorkspace  VariableName=delta_y  SaveFormat=Timeseries  SampleTime=-1
  To Workspace14 : ToWorkspace  VariableName=delta_z  SaveFormat=Timeseries  SampleTime=-1
  To Workspace2 : ToWorkspace  VariableName=Thrust  SaveFormat=Timeseries  SampleTime=-1
  Transfer Fcn : TransferFcn  Denominator=[0.5 1]
  Transfer Fcn1 : TransferFcn  Denominator=[0.5 1]
  Transfer Fcn2 : TransferFcn  Denominator=[0.01 1]
  Fthrust : Outport
  Mthrust : Outport  Port=2
  wires:
  Product2/1 -> Gain2/1
  Product1/1 -> Gain1/1
  Mux/1 -> Fthrust/1, Cross Product/2  "FTxyz"
  Cross Product/1 -> Mthrust/1
  r_xyz/1 -> Cross Product/1
  Gain1/1 -> Mux/2
  delta_z(rad)/1 -> Transfer Fcn/1
  delta_y(rad)/1 -> Transfer Fcn1/1
  Switch/1 -> To Workspace2/1, Product2/1, Product1/1, Scope/1, Mux/1
  Transfer Fcn/1 -> Angle Conversion2/1, Scope1/1, Product1/2
  Transfer Fcn1/1 -> Angle Conversion1/1, Scope1/2, Product2/2
  Gain2/1 -> Mux/3
  Tmax/1 -> Transfer Fcn2/1
  飞行阶段使能/1 -> Switch/2
  Constant/1 -> Switch/3
  Transfer Fcn2/1 -> Switch/1
  Angle Conversion2/1 -> To Workspace14/1
  Angle Conversion1/1 -> To Workspace1/1

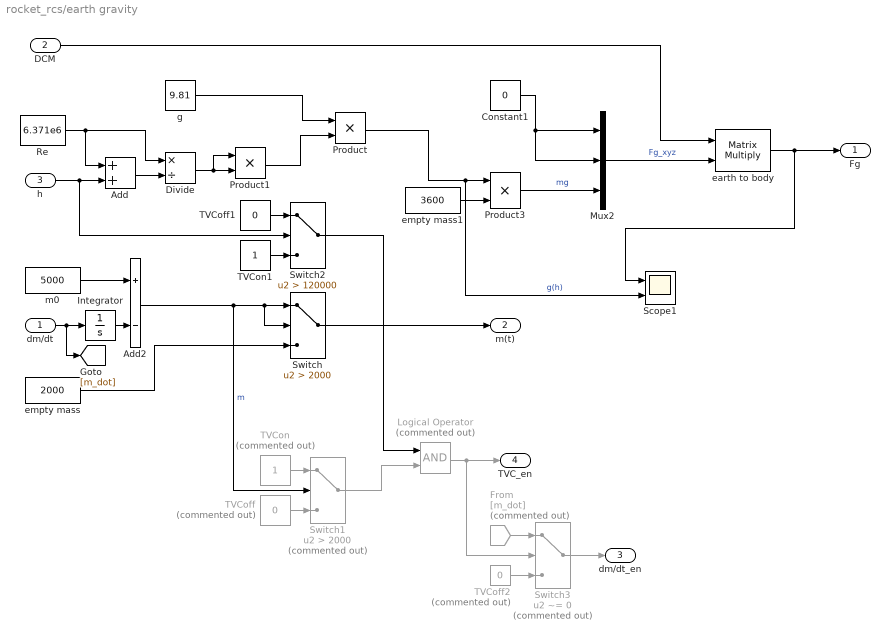
== system rocket_rcs/earth gravity ==
  dm/dt : Inport
  DCM : Inport  Port=2
  h : Inport  Port=3
  Add : Sum
  Add2 : Sum  Inputs=+-
  Constant1 : Constant  Value=0
  Divide : Product  Inputs=*/
  From : From  Commented=on  GotoTag=m_dot
  Integrator : Integrator
  Logical Operator : Logic  Commented=on  AllPortsSameDT=off  OutDataTypeStr=boolean
  Mux2 : Mux  Inputs=3
  Product : Product
  Product1 : Product
  Product3 : Product
  Re : Constant  Value=6.371e6
  Scope1 : Scope  NumInputPorts=2
  Switch : Switch  Criteria=u2 > Threshold  Threshold=2000  SaturateOnIntegerOverflow=off  InputSameDT=off
  Switch1 : Switch  Commented=on  Criteria=u2 > Threshold  Threshold=2000  SaturateOnIntegerOverflow=off  InputSameDT=off
  Switch2 : Switch  Criteria=u2 > Threshold  Threshold=120000  SaturateOnIntegerOverflow=off  InputSameDT=off
  Switch3 : Switch  Commented=on  Criteria=u2 ~= 0  SaturateOnIntegerOverflow=off  InputSameDT=off
  TVCoff : Constant  Commented=on  Value=0
  TVCoff1 : Constant  Value=0
  TVCoff2 : Constant  Commented=on  Value=0
  TVCon : Constant  Commented=on
  TVCon1 : Constant
  earth to body : Product  Multiplication=Matrix(*)
  empty mass : Constant  Value=2000
  empty mass1 : Constant  Value=3600
  g : Constant  Value=9.81
  m0 : Constant  Value=5000
  Fg : Outport
  m(t) : Outport  Port=2
  dm/dt_en : Outport  Port=3
  TVC_en : Outport  Port=4
  wires:
  Product3/1 -> Mux2/3  "mg"
  Constant1/1 -> Mux2/2, Mux2/1
  Mux2/1 -> earth to body/2  "Fg_xyz"
  dm/dt/1 -> [m_dot], Integrator/1
  m0/1 -> Add2/1
  Integrator/1 -> Add2/2
  earth to body/1 -> Scope1/1, Fg/1
  DCM/1 -> earth to body/1
  g/1 -> Product/1
  Product/1 -> Scope1/2, Product3/1  "g(h)"
  Re/1 -> Add/1, Divide/1
  Add/1 -> Divide/2
  Divide/1 -> Product1/1, Product1/2
  Product1/1 -> Product/2
  Add2/1 -> Switch1/2, Switch/2, Switch/1  "m"
  empty mass/1 -> Switch/3
  TVCon/1 -> Switch1/1
  TVCoff/1 -> Switch1/3
  Switch/1 -> m(t)/1
  Logical Operator/1 -> Switch3/2, TVC_en/1
  TVCon1/1 -> Switch2/3
  TVCoff1/1 -> Switch2/1
  h/1 -> Switch2/2, Add/2
  Switch2/1 -> Logical Operator/1
  Switch1/1 -> Logical Operator/2
  TVCoff2/1 -> Switch3/3
  From/1 -> Switch3/1
  Switch3/1 -> dm/dt_en/1
  empty mass1/1 -> Product3/2

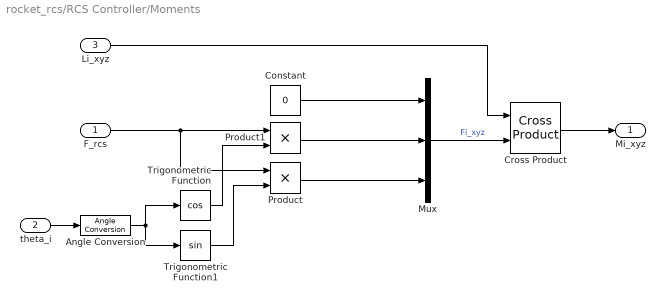
== system rocket_rcs/RCS Controller/Moments ==
  F_rcs : Inport
  theta_i : Inport  Port=2
  Li_xyz : Inport  Port=3
  Angle Conversion : aerolibconvert2/Angle Conversion  IU=deg  OU=rad
  Constant : Constant  Value=0
  Cross Product : matrix_library/Cross Product
  Mux : Mux  Inputs=3
  Product : Product
  Product1 : Product
  Trigonometric Function : Trigonometry  Operator=cos
  Trigonometric Function1 : Trigonometry
  Mi_xyz : Outport
  wires:
  Product1/1 -> Mux/2
  Product/1 -> Mux/3
  F_rcs/1 -> Product/1, Product1/1
  Trigonometric Function/1 -> Product1/2
  Trigonometric Function1/1 -> Product/2
  Constant/1 -> Mux/1
  Mux/1 -> Cross Product/2  "Fi_xyz"
  Li_xyz/1 -> Cross Product/1
  Cross Product/1 -> Mi_xyz/1
  theta_i/1 -> Angle Conversion/1
  Angle Conversion/1 -> Trigonometric Function1/1, Trigonometric Function/1

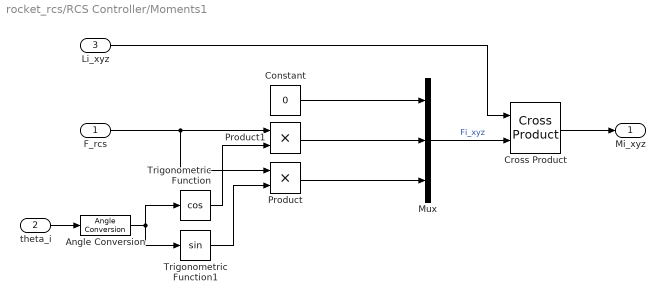
== system rocket_rcs/RCS Controller/Moments1 ==
  F_rcs : Inport
  theta_i : Inport  Port=2
  Li_xyz : Inport  Port=3
  Angle Conversion : aerolibconvert2/Angle Conversion  IU=deg  OU=rad
  Constant : Constant  Value=0
  Cross Product : matrix_library/Cross Product
  Mux : Mux  Inputs=3
  Product : Product
  Product1 : Product
  Trigonometric Function : Trigonometry  Operator=cos
  Trigonometric Function1 : Trigonometry
  Mi_xyz : Outport
  wires:
  Product1/1 -> Mux/2
  Product/1 -> Mux/3
  F_rcs/1 -> Product/1, Product1/1
  Trigonometric Function/1 -> Product1/2
  Trigonometric Function1/1 -> Product/2
  Constant/1 -> Mux/1
  Mux/1 -> Cross Product/2  "Fi_xyz"
  Li_xyz/1 -> Cross Product/1
  Cross Product/1 -> Mi_xyz/1
  theta_i/1 -> Angle Conversion/1
  Angle Conversion/1 -> Trigonometric Function1/1, Trigonometric Function/1
